simulink model "ECG_Abnormality_Analysis"  (R2026b)
settings: Solver=FixedStepDiscrete  FixedStep=1/360
values from neighbouring files (symbols this model uses):
  threshold = mean(y)+0.8*std(y)    [real_ecg_analysis.m]
libraries: simulink x1
settings Model: Creator=KiTE  LastModifiedBy=KiTE

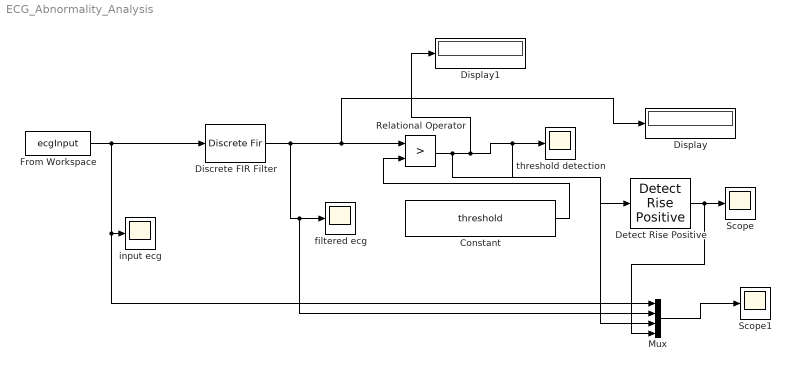
== system ECG_Abnormality_Analysis ==
  Constant : Constant  Value=threshold
  Detect Rise Positive : simulink/Logic and Bit Operations/Detect Rise Positive  vinit=0  OutDataTypeStr=boolean
  Discrete FIR Filter : DiscreteFir  Coefficients=ones(1,7)/7
  Display : Display
  Display1 : Display
  From Workspace : FromWorkspace  VariableName=ecgInput
  Mux : Mux
  Relational Operator : RelationalOperator  Operator=>  OutDataTypeStr=boolean  RndMeth=Simplest  InputSameDT=off
  Scope : Scope
      settings: ActiveDisplayYMinimum=-0.12289444311269573  ActiveDisplayYMaximum=1.0466074031524188  DataLoggingVariableName=ScopeData3
  Scope1 : Scope
      settings: DataLoggingVariableName=ScopeData4
  filtered ecg : Scope
      settings: ActiveDisplayYMinimum=7.0909032418995821  ActiveDisplayYMaximum=1348.5205953691272
  input ecg : Scope
      settings: ActiveDisplayYMinimum=7.0909032418995821  ActiveDisplayYMaximum=1348.5205953691272
  threshold detection : Scope
      settings: ActiveDisplayYMinimum=0.031600215378659764  ActiveDisplayYMaximum=0.0705602912321603  DataLoggingVariableName=ScopeData2
  wires:
  From Workspace/1 -> Mux/1, input ecg/1, Discrete FIR Filter/1
  Constant/1 -> Relational Operator/2
  Discrete FIR Filter/1 -> Mux/2, filtered ecg/1, Display/1, Relational Operator/1
  Relational Operator/1 -> Detect Rise Positive/1, Display1/1, Mux/3, threshold detection/1
  Detect Rise Positive/1 -> Mux/4, Scope/1
  Mux/1 -> Scope1/1
